simulink model "CellChannels"  (R2024a)
settings: Solver=FixedStepDiscrete  StartTime=0.0  StopTime=10  FixedStep=0.01  RelTol=1e-3
PreLoadFcn:
  | if exist('CellChannels_types', 'file') == 2, CellChannels_types(); end
model workspace (MAT data in the model file):
  CtrlKi_per_s = Simulink.Parameter
  CtrlKi_per_s.Value = 1
  CtrlKi_per_s.Complexity = 'real'
  CtrlKi_per_s.Dimensions = [1 1]
  CtrlKi_per_s.DataType = 'single'
  CtrlKp = Simulink.Parameter
  CtrlKp.Value = 0.2
  CtrlKp.Complexity = 'real'
  CtrlKp.Dimensions = [1 1]
  CtrlKp.DataType = 'single'
  CtrlLimit_V = Simulink.Parameter
  CtrlLimit_V.Value = 0.1
  CtrlLimit_V.Complexity = 'real'
  CtrlLimit_V.Dimensions = [1 1]
  CtrlLimit_V.DataType = 'single'
  OutputFloor_V = Simulink.Parameter
  OutputFloor_V.Value = 0.7
  OutputFloor_V.Complexity = 'real'
  OutputFloor_V.Dimensions = [1 1]
  OutputFloor_V.DataType = 'single'
  OverVoltThd_V = Simulink.Parameter
  OverVoltThd_V.Value = 0.2
  OverVoltThd_V.Complexity = 'real'
  OverVoltThd_V.Dimensions = [1 1]
  OverVoltThd_V.DataType = 'single'
  OverVoltTime_cycles = Simulink.Parameter
  OverVoltTime_cycles.Value = 10
  OverVoltTime_cycles.Complexity = 'real'
  OverVoltTime_cycles.Dimensions = [1 1]
  OverVoltTime_cycles.DataType = 'uint8'
  SetpointLimit_V = Simulink.Parameter
  SetpointLimit_V.Value = 5
  SetpointLimit_V.Complexity = 'real'
  SetpointLimit_V.Dimensions = [1 1]
  SetpointLimit_V.DataType = 'single'
  StepHold_cycles = Simulink.Parameter
  StepHold_cycles.Value = 50
  StepHold_cycles.Complexity = 'real'
  StepHold_cycles.Dimensions = [1 1]
  StepHold_cycles.DataType = 'uint8'
  StepThreshold_V = Simulink.Parameter
  StepThreshold_V.Value = 0.2
  StepThreshold_V.Complexity = 'real'
  StepThreshold_V.Dimensions = [1 1]
  StepThreshold_V.DataType = 'single'
  VoltageSenseFilter = Simulink.Parameter
  VoltageSenseFilter.Value = 0.1
  VoltageSenseFilter.Complexity = 'real'
  VoltageSenseFilter.Dimensions = [1 1]
  VoltageSenseFilter.DataType = 'single'
  VoltageSenseMeas_Ax = Simulink.Parameter
  VoltageSenseMeas_Ax.Value = [0 398.1 795.7 1195.8 1596.4 1996]
  VoltageSenseMeas_Ax.Complexity = 'real'
  VoltageSenseMeas_Ax.Dimensions = [1 6]
  VoltageSenseMeas_Ax.DataType = 'single'
  VoltageSenseValue_T = Simulink.Parameter
  VoltageSenseValue_T.Value = [0 1 2 3 4 5]
  VoltageSenseValue_T.Complexity = 'real'
  VoltageSenseValue_T.Dimensions = [1 6]
  VoltageSenseValue_T.DataType = 'single'
  VoltageSetPwm_T = Simulink.Parameter
  VoltageSetPwm_T.Value = [0 0.185875 0.378085 0.570892 0.763797 0.9566]
  VoltageSetPwm_T.Complexity = 'real'
  VoltageSetPwm_T.Dimensions = [1 6]
  VoltageSetPwm_T.DataType = 'single'
  VoltageSetValue_Ax = Simulink.Parameter
  VoltageSetValue_Ax.Value = [0 1 2 3 4 5]
  VoltageSetValue_Ax.Complexity = 'real'
  VoltageSetValue_Ax.Dimensions = [1 6]
  VoltageSetValue_Ax.DataType = 'single'
values from neighbouring files (symbols this model uses):
  CtrlKi_per_s = 1.0    (= 1)    [CellChannels_data.m]
  CtrlKp = 0.2    [CellChannels_data.m]
  CtrlLimit_V = 0.1    [CellChannels_data.m]
  OutputFloor_V = 0.7    [CellChannels_data.m]
  OverVoltThd_V = 0.2    [CellChannels_data.m]
  OverVoltTime_cycles = 10    [CellChannels_data.m]
  SetpointLimit_V = 5.0    (= 5)    [CellChannels_data.m]
  StepHold_cycles = 50    [CellChannels_data.m]
  StepThreshold_V = 0.2    [CellChannels_data.m]
  VoltageSenseFilter = 0.1    [CellChannels_data.m]
  VoltageSenseMeas_Ax = [0.0 398.1 795.7 1195.8 1596.4 1996.0]    [CellChannels_data.m]
  VoltageSenseValue_T = [0 1 2 3 4 5]    [CellChannels_data.m]
  VoltageSetPwm_T = [0 0.185875 0.378085 0.570892 0.763797 0.9566]    [CellChannels_data.m]
  VoltageSetValue_Ax = [0 1 2 3 4 5]    [CellChannels_data.m]
undefined symbols (not defined in the file or in its folder): QLF_OK
Description:
  | 14 Zellkanaele: Sollwert auf Tastgrad, Freigabe, Istwert, Kalibrierung, Regler und Status
settings Model: ParameterArgumentNames=VoltageSetValue_Ax,VoltageSetPwm_T,VoltageSenseMeas_Ax,VoltageSenseValue_T,SetpointLimit_V,OverVoltThd_V,OverVoltTime_cycles,OutputFloor_V,StepThreshold_V,StepHold_cycles,VoltageSenseFilter,CtrlKp,CtrlKi_per_s,CtrlLimit_V  Creator=danie  LastModifiedBy=danie
settings OptimizationCC: DefaultParameterBehavior=Inlined  EnhancedBackFolding=on  PassReuseOutputArgsAs=Individual arguments  ZeroExternalMemoryAtStartup=off  ZeroInternalMemoryAtStartup=off  OptimizeBlockOrder=speed  DifferentSizesBufferReuse=on  OptimizationCustomize=off  EfficientTunableParamExpr=on
settings DebuggingCC: ParameterTunabilityLossMsg=error
settings HardwareCC: ProdBitPerPointer=32  ProdBitPerSizeT=32  ProdBitPerPtrDiffT=32  ProdLargestAtomicInteger=Long  ProdLargestAtomicFloat=Double  ProdWordSize=32  ProdLongLongMode=on  ProdHWDeviceType=ARM Compatible->ARM Cortex-M
settings SFSimCC: MATLABDynamicMemAlloc=off
settings RTWCC: Description=AUTOSAR  SystemTargetFile=autosar.tlc  GenCodeOnly=on  GenerateMakefile=off  TemplateMakefile=ert_default_tmf  DataTypeReplacement=CDataTypesFixedWidth
settings CodeAppCC: ForceParamTrailComments=on  IgnoreCustomStorageClasses=off  MaxIdLength=63  OperatorAnnotations=on  SimulinkDataObjDesc=on  SFDataObjDesc=on  InsertBlockDesc=on
settings STFCustomTargetCC: MultiwordLength=256  ParMdlRefBuildCompliant=on  CompOptLevelCompliant=on  IncludeMdlTerminateFcn=off  CombineOutputUpdateFcns=on  SuppressErrorStatus=on  ERTCustomFileBanners=on  SupportNonFinite=off  SupportComplex=off  SupportContinuousTime=off  SupportNonInlinedSFcns=off  RemoveResetFunc=on  MATLABClassNameForMDSCustomization=Simulink.SoftwareTarget.ERTCustomization  AutosarCompliant=on  GRTInterface=off  LookupTableObjectStructAxisOrder=2,1,3,4,...  LUTObjectStructOrderEvenSpacing=Size,Table,Breakpoints  SystemTargetFile=autosar.tlc
settings ERTTargetCC: TargetLangStandard=C99 (ISO)  ConcurrentExecutionCompliant=off  IncludeMdlTerminateFcn=off  SuppressErrorStatus=on  SupportNonFinite=off  SupportComplex=off  ModelStepFunctionPrototypeControlCompliant=off  CPPClassGenCompliant=off  AutosarCompliant=on  LookupTableObjectStructAxisOrder=2,1,3,4,...  LUTObjectStructOrderEvenSpacing=Size,Table,Breakpoints  InlinedParameterPlacement=NonHierarchical  ERTCustomFileTemplate=example_file_process.tlc  BooleanTrueId=TRUE  BooleanFalseId=FALSE

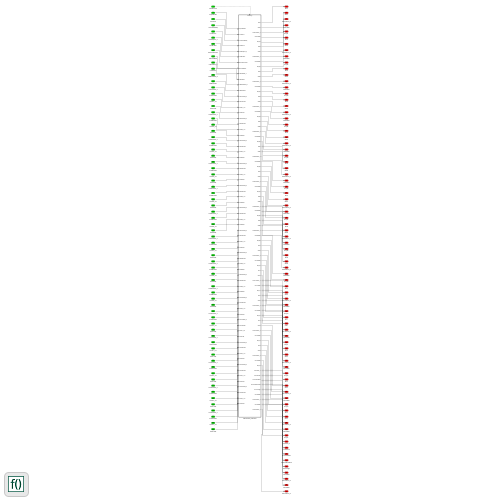
[thumbnail: Simulink's stored preview of the top-level diagram]
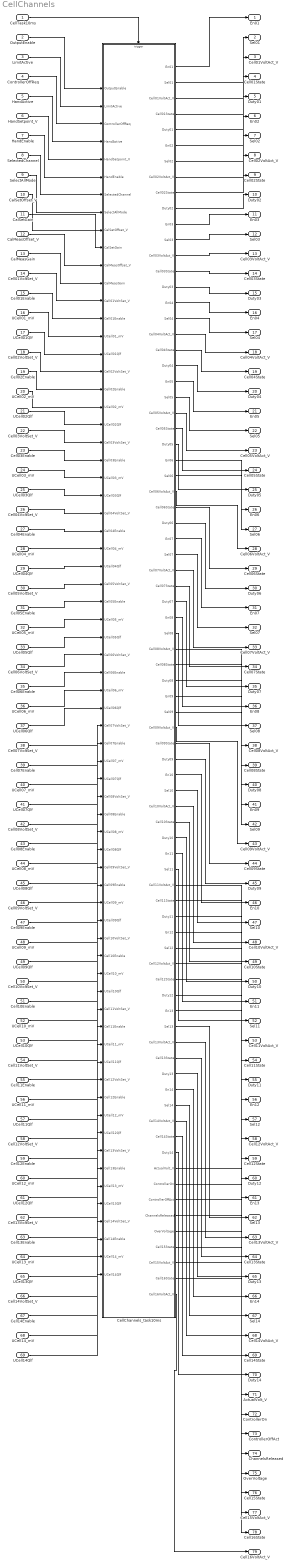
== system CellChannels ==
  CellTask10ms : Inport  SampleTime=0.01  OutputFunctionCall=on
  OutputEnable : Inport  Port=2  OutDataTypeStr=boolean  PortDimensions=1
  LimitActive : Inport  Port=3  OutDataTypeStr=boolean  PortDimensions=1
  ControllerOffReq : Inport  Port=4  OutDataTypeStr=uint8  PortDimensions=1
  HandActive : Inport  Port=5  OutDataTypeStr=boolean  PortDimensions=1
  HandSetpoint_V : Inport  Port=6  OutDataTypeStr=single  PortDimensions=CellCount
  HandEnable : Inport  Port=7  OutDataTypeStr=boolean  PortDimensions=CellCount
  SelectedChannel : Inport  Port=8  OutDataTypeStr=uint8  PortDimensions=1
  SelectAllMode : Inport  Port=9  OutDataTypeStr=boolean  PortDimensions=1
  CalSetOffset_V : Inport  Port=10  OutDataTypeStr=single  PortDimensions=CellCount
  CalSetGain : Inport  Port=11  OutDataTypeStr=single  PortDimensions=CellCount
  CalMeasOffset_V : Inport  Port=12  OutDataTypeStr=single  PortDimensions=CellCount
  CalMeasGain : Inport  Port=13  OutDataTypeStr=single  PortDimensions=CellCount
  Cell01VoltSet_V : Inport  Port=14  OutDataTypeStr=single  PortDimensions=1
  Cell01Enable : Inport  Port=15  OutDataTypeStr=uint8  PortDimensions=1
  UCell01_mV : Inport  Port=16  OutDataTypeStr=uint32  PortDimensions=1
  UCell01Qlf : Inport  Port=17  OutDataTypeStr=uint8  PortDimensions=1
  Cell02VoltSet_V : Inport  Port=18  OutDataTypeStr=single  PortDimensions=1
  Cell02Enable : Inport  Port=19  OutDataTypeStr=uint8  PortDimensions=1
  UCell02_mV : Inport  Port=20  OutDataTypeStr=uint32  PortDimensions=1
  UCell02Qlf : Inport  Port=21  OutDataTypeStr=uint8  PortDimensions=1
  Cell03VoltSet_V : Inport  Port=22  OutDataTypeStr=single  PortDimensions=1
  Cell03Enable : Inport  Port=23  OutDataTypeStr=uint8  PortDimensions=1
  UCell03_mV : Inport  Port=24  OutDataTypeStr=uint32  PortDimensions=1
  UCell03Qlf : Inport  Port=25  OutDataTypeStr=uint8  PortDimensions=1
  Cell04VoltSet_V : Inport  Port=26  OutDataTypeStr=single  PortDimensions=1
  Cell04Enable : Inport  Port=27  OutDataTypeStr=uint8  PortDimensions=1
  UCell04_mV : Inport  Port=28  OutDataTypeStr=uint32  PortDimensions=1
  UCell04Qlf : Inport  Port=29  OutDataTypeStr=uint8  PortDimensions=1
  Cell05VoltSet_V : Inport  Port=30  OutDataTypeStr=single  PortDimensions=1
  Cell05Enable : Inport  Port=31  OutDataTypeStr=uint8  PortDimensions=1
  UCell05_mV : Inport  Port=32  OutDataTypeStr=uint32  PortDimensions=1
  UCell05Qlf : Inport  Port=33  OutDataTypeStr=uint8  PortDimensions=1
  Cell06VoltSet_V : Inport  Port=34  OutDataTypeStr=single  PortDimensions=1
  Cell06Enable : Inport  Port=35  OutDataTypeStr=uint8  PortDimensions=1
  UCell06_mV : Inport  Port=36  OutDataTypeStr=uint32  PortDimensions=1
  UCell06Qlf : Inport  Port=37  OutDataTypeStr=uint8  PortDimensions=1
  Cell07VoltSet_V : Inport  Port=38  OutDataTypeStr=single  PortDimensions=1
  Cell07Enable : Inport  Port=39  OutDataTypeStr=uint8  PortDimensions=1
  UCell07_mV : Inport  Port=40  OutDataTypeStr=uint32  PortDimensions=1
  UCell07Qlf : Inport  Port=41  OutDataTypeStr=uint8  PortDimensions=1
  Cell08VoltSet_V : Inport  Port=42  OutDataTypeStr=single  PortDimensions=1
  Cell08Enable : Inport  Port=43  OutDataTypeStr=uint8  PortDimensions=1
  UCell08_mV : Inport  Port=44  OutDataTypeStr=uint32  PortDimensions=1
  UCell08Qlf : Inport  Port=45  OutDataTypeStr=uint8  PortDimensions=1
  Cell09VoltSet_V : Inport  Port=46  OutDataTypeStr=single  PortDimensions=1
  Cell09Enable : Inport  Port=47  OutDataTypeStr=uint8  PortDimensions=1
  UCell09_mV : Inport  Port=48  OutDataTypeStr=uint32  PortDimensions=1
  UCell09Qlf : Inport  Port=49  OutDataTypeStr=uint8  PortDimensions=1
  Cell10VoltSet_V : Inport  Port=50  OutDataTypeStr=single  PortDimensions=1
  Cell10Enable : Inport  Port=51  OutDataTypeStr=uint8  PortDimensions=1
  UCell10_mV : Inport  Port=52  OutDataTypeStr=uint32  PortDimensions=1
  UCell10Qlf : Inport  Port=53  OutDataTypeStr=uint8  PortDimensions=1
  Cell11VoltSet_V : Inport  Port=54  OutDataTypeStr=single  PortDimensions=1
  Cell11Enable : Inport  Port=55  OutDataTypeStr=uint8  PortDimensions=1
  UCell11_mV : Inport  Port=56  OutDataTypeStr=uint32  PortDimensions=1
  UCell11Qlf : Inport  Port=57  OutDataTypeStr=uint8  PortDimensions=1
  Cell12VoltSet_V : Inport  Port=58  OutDataTypeStr=single  PortDimensions=1
  Cell12Enable : Inport  Port=59  OutDataTypeStr=uint8  PortDimensions=1
  UCell12_mV : Inport  Port=60  OutDataTypeStr=uint32  PortDimensions=1
  UCell12Qlf : Inport  Port=61  OutDataTypeStr=uint8  PortDimensions=1
  Cell13VoltSet_V : Inport  Port=62  OutDataTypeStr=single  PortDimensions=1
  Cell13Enable : Inport  Port=63  OutDataTypeStr=uint8  PortDimensions=1
  UCell13_mV : Inport  Port=64  OutDataTypeStr=uint32  PortDimensions=1
  UCell13Qlf : Inport  Port=65  OutDataTypeStr=uint8  PortDimensions=1
  Cell14VoltSet_V : Inport  Port=66  OutDataTypeStr=single  PortDimensions=1
  Cell14Enable : Inport  Port=67  OutDataTypeStr=uint8  PortDimensions=1
  UCell14_mV : Inport  Port=68  OutDataTypeStr=uint32  PortDimensions=1
  UCell14Qlf : Inport  Port=69  OutDataTypeStr=uint8  PortDimensions=1
  CellChannels_task10ms : Subsystem  TreatAsAtomicUnit=on
  En01 : Outport  OutDataTypeStr=boolean  PortDimensions=1
  Sel01 : Outport  Port=2  OutDataTypeStr=boolean  PortDimensions=1
  Cell01VoltAct_V : Outport  Port=3  OutDataTypeStr=single  PortDimensions=1
  Cell01State : Outport  Port=4  OutDataTypeStr=uint8  PortDimensions=1
  Duty01 : Outport  Port=5  OutDataTypeStr=uint16  PortDimensions=1
  En02 : Outport  Port=6  OutDataTypeStr=boolean  PortDimensions=1
  Sel02 : Outport  Port=7  OutDataTypeStr=boolean  PortDimensions=1
  Cell02VoltAct_V : Outport  Port=8  OutDataTypeStr=single  PortDimensions=1
  Cell02State : Outport  Port=9  OutDataTypeStr=uint8  PortDimensions=1
  Duty02 : Outport  Port=10  OutDataTypeStr=uint16  PortDimensions=1
  En03 : Outport  Port=11  OutDataTypeStr=boolean  PortDimensions=1
  Sel03 : Outport  Port=12  OutDataTypeStr=boolean  PortDimensions=1
  Cell03VoltAct_V : Outport  Port=13  OutDataTypeStr=single  PortDimensions=1
  Cell03State : Outport  Port=14  OutDataTypeStr=uint8  PortDimensions=1
  Duty03 : Outport  Port=15  OutDataTypeStr=uint16  PortDimensions=1
  En04 : Outport  Port=16  OutDataTypeStr=boolean  PortDimensions=1
  Sel04 : Outport  Port=17  OutDataTypeStr=boolean  PortDimensions=1
  Cell04VoltAct_V : Outport  Port=18  OutDataTypeStr=single  PortDimensions=1
  Cell04State : Outport  Port=19  OutDataTypeStr=uint8  PortDimensions=1
  Duty04 : Outport  Port=20  OutDataTypeStr=uint16  PortDimensions=1
  En05 : Outport  Port=21  OutDataTypeStr=boolean  PortDimensions=1
  Sel05 : Outport  Port=22  OutDataTypeStr=boolean  PortDimensions=1
  Cell05VoltAct_V : Outport  Port=23  OutDataTypeStr=single  PortDimensions=1
  Cell05State : Outport  Port=24  OutDataTypeStr=uint8  PortDimensions=1
  Duty05 : Outport  Port=25  OutDataTypeStr=uint16  PortDimensions=1
  En06 : Outport  Port=26  OutDataTypeStr=boolean  PortDimensions=1
  Sel06 : Outport  Port=27  OutDataTypeStr=boolean  PortDimensions=1
  Cell06VoltAct_V : Outport  Port=28  OutDataTypeStr=single  PortDimensions=1
  Cell06State : Outport  Port=29  OutDataTypeStr=uint8  PortDimensions=1
  Duty06 : Outport  Port=30  OutDataTypeStr=uint16  PortDimensions=1
  En07 : Outport  Port=31  OutDataTypeStr=boolean  PortDimensions=1
  Sel07 : Outport  Port=32  OutDataTypeStr=boolean  PortDimensions=1
  Cell07VoltAct_V : Outport  Port=33  OutDataTypeStr=single  PortDimensions=1
  Cell07State : Outport  Port=34  OutDataTypeStr=uint8  PortDimensions=1
  Duty07 : Outport  Port=35  OutDataTypeStr=uint16  PortDimensions=1
  En08 : Outport  Port=36  OutDataTypeStr=boolean  PortDimensions=1
  Sel08 : Outport  Port=37  OutDataTypeStr=boolean  PortDimensions=1
  Cell08VoltAct_V : Outport  Port=38  OutDataTypeStr=single  PortDimensions=1
  Cell08State : Outport  Port=39  OutDataTypeStr=uint8  PortDimensions=1
  Duty08 : Outport  Port=40  OutDataTypeStr=uint16  PortDimensions=1
  En09 : Outport  Port=41  OutDataTypeStr=boolean  PortDimensions=1
  Sel09 : Outport  Port=42  OutDataTypeStr=boolean  PortDimensions=1
  Cell09VoltAct_V : Outport  Port=43  OutDataTypeStr=single  PortDimensions=1
  Cell09State : Outport  Port=44  OutDataTypeStr=uint8  PortDimensions=1
  Duty09 : Outport  Port=45  OutDataTypeStr=uint16  PortDimensions=1
  En10 : Outport  Port=46  OutDataTypeStr=boolean  PortDimensions=1
  Sel10 : Outport  Port=47  OutDataTypeStr=boolean  PortDimensions=1
  Cell10VoltAct_V : Outport  Port=48  OutDataTypeStr=single  PortDimensions=1
  Cell10State : Outport  Port=49  OutDataTypeStr=uint8  PortDimensions=1
  Duty10 : Outport  Port=50  OutDataTypeStr=uint16  PortDimensions=1
  En11 : Outport  Port=51  OutDataTypeStr=boolean  PortDimensions=1
  Sel11 : Outport  Port=52  OutDataTypeStr=boolean  PortDimensions=1
  Cell11VoltAct_V : Outport  Port=53  OutDataTypeStr=single  PortDimensions=1
  Cell11State : Outport  Port=54  OutDataTypeStr=uint8  PortDimensions=1
  Duty11 : Outport  Port=55  OutDataTypeStr=uint16  PortDimensions=1
  En12 : Outport  Port=56  OutDataTypeStr=boolean  PortDimensions=1
  Sel12 : Outport  Port=57  OutDataTypeStr=boolean  PortDimensions=1
  Cell12VoltAct_V : Outport  Port=58  OutDataTypeStr=single  PortDimensions=1
  Cell12State : Outport  Port=59  OutDataTypeStr=uint8  PortDimensions=1
  Duty12 : Outport  Port=60  OutDataTypeStr=uint16  PortDimensions=1
  En13 : Outport  Port=61  OutDataTypeStr=boolean  PortDimensions=1
  Sel13 : Outport  Port=62  OutDataTypeStr=boolean  PortDimensions=1
  Cell13VoltAct_V : Outport  Port=63  OutDataTypeStr=single  PortDimensions=1
  Cell13State : Outport  Port=64  OutDataTypeStr=uint8  PortDimensions=1
  Duty13 : Outport  Port=65  OutDataTypeStr=uint16  PortDimensions=1
  En14 : Outport  Port=66  OutDataTypeStr=boolean  PortDimensions=1
  Sel14 : Outport  Port=67  OutDataTypeStr=boolean  PortDimensions=1
  Cell14VoltAct_V : Outport  Port=68  OutDataTypeStr=single  PortDimensions=1
  Cell14State : Outport  Port=69  OutDataTypeStr=uint8  PortDimensions=1
  Duty14 : Outport  Port=70  OutDataTypeStr=uint16  PortDimensions=1
  ActualVolt_V : Outport  Port=71  OutDataTypeStr=single  PortDimensions=CellCount
  ControllerOn : Outport  Port=72  OutDataTypeStr=boolean  PortDimensions=1
  ControllerOffAct : Outport  Port=73  OutDataTypeStr=uint8  PortDimensions=1
  ChannelsReleased : Outport  Port=74  OutDataTypeStr=boolean  PortDimensions=1
  OverVoltage : Outport  Port=75  OutDataTypeStr=boolean  PortDimensions=1
  Cell15State : Outport  Port=76  OutDataTypeStr=uint8  PortDimensions=1
  Cell15VoltAct_V : Outport  Port=77  OutDataTypeStr=single  PortDimensions=1
  Cell16State : Outport  Port=78  OutDataTypeStr=uint8  PortDimensions=1
  Cell16VoltAct_V : Outport  Port=79  OutDataTypeStr=single  PortDimensions=1
  wires:
  CellTask10ms/1 -> CellChannels_task10ms/Trigger
  OutputEnable/1 -> CellChannels_task10ms/1(OutputEnable)
  LimitActive/1 -> CellChannels_task10ms/2(LimitActive)
  ControllerOffReq/1 -> CellChannels_task10ms/3(ControllerOffReq)
  HandActive/1 -> CellChannels_task10ms/4(HandActive)
  HandSetpoint_V/1 -> CellChannels_task10ms/5(HandSetpoint_V)
  HandEnable/1 -> CellChannels_task10ms/6(HandEnable)
  SelectedChannel/1 -> CellChannels_task10ms/7(SelectedChannel)
  SelectAllMode/1 -> CellChannels_task10ms/8(SelectAllMode)
  CalSetOffset_V/1 -> CellChannels_task10ms/9(CalSetOffset_V)
  CalSetGain/1 -> CellChannels_task10ms/10(CalSetGain)
  CalMeasOffset_V/1 -> CellChannels_task10ms/11(CalMeasOffset_V)
  CalMeasGain/1 -> CellChannels_task10ms/12(CalMeasGain)
  Cell01VoltSet_V/1 -> CellChannels_task10ms/13(Cell01VoltSet_V)
  Cell01Enable/1 -> CellChannels_task10ms/14(Cell01Enable)
  UCell01_mV/1 -> CellChannels_task10ms/15(UCell01_mV)
  UCell01Qlf/1 -> CellChannels_task10ms/16(UCell01Qlf)
  Cell02VoltSet_V/1 -> CellChannels_task10ms/17(Cell02VoltSet_V)
  Cell02Enable/1 -> CellChannels_task10ms/18(Cell02Enable)
  UCell02_mV/1 -> CellChannels_task10ms/19(UCell02_mV)
  UCell02Qlf/1 -> CellChannels_task10ms/20(UCell02Qlf)
  Cell03VoltSet_V/1 -> CellChannels_task10ms/21(Cell03VoltSet_V)
  Cell03Enable/1 -> CellChannels_task10ms/22(Cell03Enable)
  UCell03_mV/1 -> CellChannels_task10ms/23(UCell03_mV)
  UCell03Qlf/1 -> CellChannels_task10ms/24(UCell03Qlf)
  Cell04VoltSet_V/1 -> CellChannels_task10ms/25(Cell04VoltSet_V)
  Cell04Enable/1 -> CellChannels_task10ms/26(Cell04Enable)
  UCell04_mV/1 -> CellChannels_task10ms/27(UCell04_mV)
  UCell04Qlf/1 -> CellChannels_task10ms/28(UCell04Qlf)
  Cell05VoltSet_V/1 -> CellChannels_task10ms/29(Cell05VoltSet_V)
  Cell05Enable/1 -> CellChannels_task10ms/30(Cell05Enable)
  UCell05_mV/1 -> CellChannels_task10ms/31(UCell05_mV)
  UCell05Qlf/1 -> CellChannels_task10ms/32(UCell05Qlf)
  Cell06VoltSet_V/1 -> CellChannels_task10ms/33(Cell06VoltSet_V)
  Cell06Enable/1 -> CellChannels_task10ms/34(Cell06Enable)
  UCell06_mV/1 -> CellChannels_task10ms/35(UCell06_mV)
  UCell06Qlf/1 -> CellChannels_task10ms/36(UCell06Qlf)
  Cell07VoltSet_V/1 -> CellChannels_task10ms/37(Cell07VoltSet_V)
  Cell07Enable/1 -> CellChannels_task10ms/38(Cell07Enable)
  UCell07_mV/1 -> CellChannels_task10ms/39(UCell07_mV)
  UCell07Qlf/1 -> CellChannels_task10ms/40(UCell07Qlf)
  Cell08VoltSet_V/1 -> CellChannels_task10ms/41(Cell08VoltSet_V)
  Cell08Enable/1 -> CellChannels_task10ms/42(Cell08Enable)
  UCell08_mV/1 -> CellChannels_task10ms/43(UCell08_mV)
  UCell08Qlf/1 -> CellChannels_task10ms/44(UCell08Qlf)
  Cell09VoltSet_V/1 -> CellChannels_task10ms/45(Cell09VoltSet_V)
  Cell09Enable/1 -> CellChannels_task10ms/46(Cell09Enable)
  UCell09_mV/1 -> CellChannels_task10ms/47(UCell09_mV)
  UCell09Qlf/1 -> CellChannels_task10ms/48(UCell09Qlf)
  Cell10VoltSet_V/1 -> CellChannels_task10ms/49(Cell10VoltSet_V)
  Cell10Enable/1 -> CellChannels_task10ms/50(Cell10Enable)
  UCell10_mV/1 -> CellChannels_task10ms/51(UCell10_mV)
  UCell10Qlf/1 -> CellChannels_task10ms/52(UCell10Qlf)
  Cell11VoltSet_V/1 -> CellChannels_task10ms/53(Cell11VoltSet_V)
  Cell11Enable/1 -> CellChannels_task10ms/54(Cell11Enable)
  UCell11_mV/1 -> CellChannels_task10ms/55(UCell11_mV)
  UCell11Qlf/1 -> CellChannels_task10ms/56(UCell11Qlf)
  Cell12VoltSet_V/1 -> CellChannels_task10ms/57(Cell12VoltSet_V)
  Cell12Enable/1 -> CellChannels_task10ms/58(Cell12Enable)
  UCell12_mV/1 -> CellChannels_task10ms/59(UCell12_mV)
  UCell12Qlf/1 -> CellChannels_task10ms/60(UCell12Qlf)
  Cell13VoltSet_V/1 -> CellChannels_task10ms/61(Cell13VoltSet_V)
  Cell13Enable/1 -> CellChannels_task10ms/62(Cell13Enable)
  UCell13_mV/1 -> CellChannels_task10ms/63(UCell13_mV)
  UCell13Qlf/1 -> CellChannels_task10ms/64(UCell13Qlf)
  Cell14VoltSet_V/1 -> CellChannels_task10ms/65(Cell14VoltSet_V)
  Cell14Enable/1 -> CellChannels_task10ms/66(Cell14Enable)
  UCell14_mV/1 -> CellChannels_task10ms/67(UCell14_mV)
  UCell14Qlf/1 -> CellChannels_task10ms/68(UCell14Qlf)
  CellChannels_task10ms/1(En01) -> En01/1
  CellChannels_task10ms/2(Sel01) -> Sel01/1
  CellChannels_task10ms/3(Cell01VoltAct_V) -> Cell01VoltAct_V/1
  CellChannels_task10ms/4(Cell01State) -> Cell01State/1
  CellChannels_task10ms/5(Duty01) -> Duty01/1
  CellChannels_task10ms/6(En02) -> En02/1
  CellChannels_task10ms/7(Sel02) -> Sel02/1
  CellChannels_task10ms/8(Cell02VoltAct_V) -> Cell02VoltAct_V/1
  CellChannels_task10ms/9(Cell02State) -> Cell02State/1
  CellChannels_task10ms/10(Duty02) -> Duty02/1
  CellChannels_task10ms/11(En03) -> En03/1
  CellChannels_task10ms/12(Sel03) -> Sel03/1
  CellChannels_task10ms/13(Cell03VoltAct_V) -> Cell03VoltAct_V/1
  CellChannels_task10ms/14(Cell03State) -> Cell03State/1
  CellChannels_task10ms/15(Duty03) -> Duty03/1
  CellChannels_task10ms/16(En04) -> En04/1
  CellChannels_task10ms/17(Sel04) -> Sel04/1
  CellChannels_task10ms/18(Cell04VoltAct_V) -> Cell04VoltAct_V/1
  CellChannels_task10ms/19(Cell04State) -> Cell04State/1
  CellChannels_task10ms/20(Duty04) -> Duty04/1
  CellChannels_task10ms/21(En05) -> En05/1
  CellChannels_task10ms/22(Sel05) -> Sel05/1
  CellChannels_task10ms/23(Cell05VoltAct_V) -> Cell05VoltAct_V/1
  CellChannels_task10ms/24(Cell05State) -> Cell05State/1
  CellChannels_task10ms/25(Duty05) -> Duty05/1
  CellChannels_task10ms/26(En06) -> En06/1
  CellChannels_task10ms/27(Sel06) -> Sel06/1
  CellChannels_task10ms/28(Cell06VoltAct_V) -> Cell06VoltAct_V/1
  CellChannels_task10ms/29(Cell06State) -> Cell06State/1
  CellChannels_task10ms/30(Duty06) -> Duty06/1
  CellChannels_task10ms/31(En07) -> En07/1
  CellChannels_task10ms/32(Sel07) -> Sel07/1
  CellChannels_task10ms/33(Cell07VoltAct_V) -> Cell07VoltAct_V/1
  CellChannels_task10ms/34(Cell07State) -> Cell07State/1
  CellChannels_task10ms/35(Duty07) -> Duty07/1
  CellChannels_task10ms/36(En08) -> En08/1
  CellChannels_task10ms/37(Sel08) -> Sel08/1
  CellChannels_task10ms/38(Cell08VoltAct_V) -> Cell08VoltAct_V/1
  CellChannels_task10ms/39(Cell08State) -> Cell08State/1
  CellChannels_task10ms/40(Duty08) -> Duty08/1
  CellChannels_task10ms/41(En09) -> En09/1
  CellChannels_task10ms/42(Sel09) -> Sel09/1
  CellChannels_task10ms/43(Cell09VoltAct_V) -> Cell09VoltAct_V/1
  CellChannels_task10ms/44(Cell09State) -> Cell09State/1
  CellChannels_task10ms/45(Duty09) -> Duty09/1
  CellChannels_task10ms/46(En10) -> En10/1
  CellChannels_task10ms/47(Sel10) -> Sel10/1
  CellChannels_task10ms/48(Cell10VoltAct_V) -> Cell10VoltAct_V/1
  CellChannels_task10ms/49(Cell10State) -> Cell10State/1
  CellChannels_task10ms/50(Duty10) -> Duty10/1
  CellChannels_task10ms/51(En11) -> En11/1
  CellChannels_task10ms/52(Sel11) -> Sel11/1
  CellChannels_task10ms/53(Cell11VoltAct_V) -> Cell11VoltAct_V/1
  CellChannels_task10ms/54(Cell11State) -> Cell11State/1
  CellChannels_task10ms/55(Duty11) -> Duty11/1
  CellChannels_task10ms/56(En12) -> En12/1
  CellChannels_task10ms/57(Sel12) -> Sel12/1
  CellChannels_task10ms/58(Cell12VoltAct_V) -> Cell12VoltAct_V/1
  CellChannels_task10ms/59(Cell12State) -> Cell12State/1
  CellChannels_task10ms/60(Duty12) -> Duty12/1
  CellChannels_task10ms/61(En13) -> En13/1
  CellChannels_task10ms/62(Sel13) -> Sel13/1
  CellChannels_task10ms/63(Cell13VoltAct_V) -> Cell13VoltAct_V/1
  CellChannels_task10ms/64(Cell13State) -> Cell13State/1
  CellChannels_task10ms/65(Duty13) -> Duty13/1
  CellChannels_task10ms/66(En14) -> En14/1
  CellChannels_task10ms/67(Sel14) -> Sel14/1
  CellChannels_task10ms/68(Cell14VoltAct_V) -> Cell14VoltAct_V/1
  CellChannels_task10ms/69(Cell14State) -> Cell14State/1
  CellChannels_task10ms/70(Duty14) -> Duty14/1
  CellChannels_task10ms/71(ActualVolt_V) -> ActualVolt_V/1
  CellChannels_task10ms/72(ControllerOn) -> ControllerOn/1
  CellChannels_task10ms/73(ControllerOffAct) -> ControllerOffAct/1
  CellChannels_task10ms/74(ChannelsReleased) -> ChannelsReleased/1
  CellChannels_task10ms/75(OverVoltage) -> OverVoltage/1
  CellChannels_task10ms/76(Cell15State) -> Cell15State/1
  CellChannels_task10ms/77(Cell15VoltAct_V) -> Cell15VoltAct_V/1
  CellChannels_task10ms/78(Cell16State) -> Cell16State/1
  CellChannels_task10ms/79(Cell16VoltAct_V) -> Cell16VoltAct_V/1

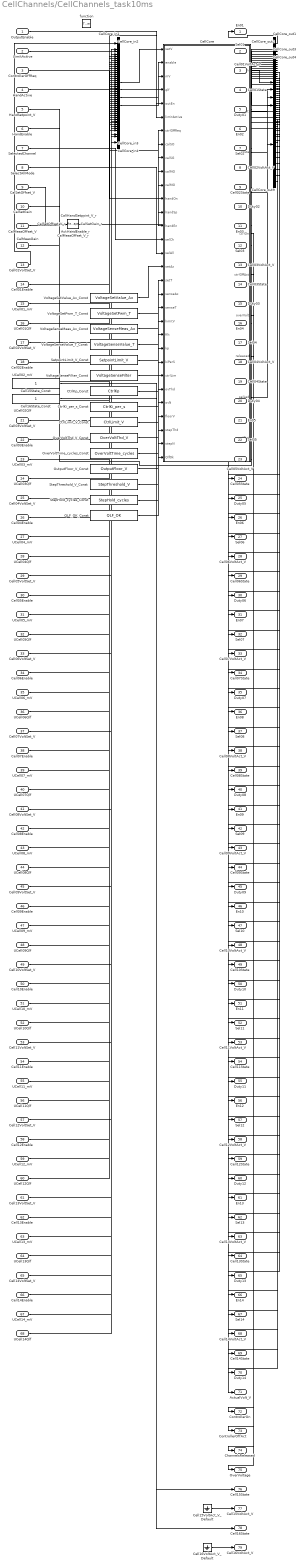
== system CellChannels/CellChannels_task10ms ==
  OutputEnable : Inport
  LimitActive : Inport  Port=2
  ControllerOffReq : Inport  Port=3
  HandActive : Inport  Port=4
  HandSetpoint_V : Inport  Port=5
  HandEnable : Inport  Port=6
  SelectedChannel : Inport  Port=7
  SelectAllMode : Inport  Port=8
  CalSetOffset_V : Inport  Port=9
  CalSetGain : Inport  Port=10
  CalMeasOffset_V : Inport  Port=11
  CalMeasGain : Inport  Port=12
  Cell01VoltSet_V : Inport  Port=13
  Cell01Enable : Inport  Port=14
  UCell01_mV : Inport  Port=15
  UCell01Qlf : Inport  Port=16
  Cell02VoltSet_V : Inport  Port=17
  Cell02Enable : Inport  Port=18
  UCell02_mV : Inport  Port=19
  UCell02Qlf : Inport  Port=20
  Cell03VoltSet_V : Inport  Port=21
  Cell03Enable : Inport  Port=22
  UCell03_mV : Inport  Port=23
  UCell03Qlf : Inport  Port=24
  Cell04VoltSet_V : Inport  Port=25
  Cell04Enable : Inport  Port=26
  UCell04_mV : Inport  Port=27
  UCell04Qlf : Inport  Port=28
  Cell05VoltSet_V : Inport  Port=29
  Cell05Enable : Inport  Port=30
  UCell05_mV : Inport  Port=31
  UCell05Qlf : Inport  Port=32
  Cell06VoltSet_V : Inport  Port=33
  Cell06Enable : Inport  Port=34
  UCell06_mV : Inport  Port=35
  UCell06Qlf : Inport  Port=36
  Cell07VoltSet_V : Inport  Port=37
  Cell07Enable : Inport  Port=38
  UCell07_mV : Inport  Port=39
  UCell07Qlf : Inport  Port=40
  Cell08VoltSet_V : Inport  Port=41
  Cell08Enable : Inport  Port=42
  UCell08_mV : Inport  Port=43
  UCell08Qlf : Inport  Port=44
  Cell09VoltSet_V : Inport  Port=45
  Cell09Enable : Inport  Port=46
  UCell09_mV : Inport  Port=47
  UCell09Qlf : Inport  Port=48
  Cell10VoltSet_V : Inport  Port=49
  Cell10Enable : Inport  Port=50
  UCell10_mV : Inport  Port=51
  UCell10Qlf : Inport  Port=52
  Cell11VoltSet_V : Inport  Port=53
  Cell11Enable : Inport  Port=54
  UCell11_mV : Inport  Port=55
  UCell11Qlf : Inport  Port=56
  Cell12VoltSet_V : Inport  Port=57
  Cell12Enable : Inport  Port=58
  UCell12_mV : Inport  Port=59
  UCell12Qlf : Inport  Port=60
  Cell13VoltSet_V : Inport  Port=61
  Cell13Enable : Inport  Port=62
  UCell13_mV : Inport  Port=63
  UCell13Qlf : Inport  Port=64
  Cell14VoltSet_V : Inport  Port=65
  Cell14Enable : Inport  Port=66
  UCell14_mV : Inport  Port=67
  UCell14Qlf : Inport  Port=68
  function : TriggerPort  TriggerType=function-call  VariantControl=(inherit)  SampleTimeType=periodic  SampleTime=0.01
  ActualVolt_V_r : Reshape
  CalMeasGain_r : Reshape  OutputDimensionality=Customize  OutputDimensions=[14 1]
  CalMeasOffset_V_r : Reshape  OutputDimensionality=Customize  OutputDimensions=[14 1]
  CalSetGain_r : Reshape  OutputDimensionality=Customize  OutputDimensions=[14 1]
  CalSetOffset_V_r : Reshape  OutputDimensionality=Customize  OutputDimensions=[14 1]
  Cell15State_Const : Constant  OutDataTypeStr=uint8
  Cell15VoltAct_V_Default : Ground
  Cell16State_Const : Constant  OutDataTypeStr=uint8
  Cell16VoltAct_V_Default : Ground
  CellCore : MATLAB Function  TreatAsAtomicUnit=on
  CellCore_in{1..4} (4 alike) : Mux  Inputs=14
  CellCore_out{1..4,9} (5 alike) : Demux  Outputs=14
  CtrlKi_per_s_Const : Constant  Value=CtrlKi_per_s  OutDataTypeStr=single
  CtrlKp_Const : Constant  Value=CtrlKp  OutDataTypeStr=single
  CtrlLimit_V_Const : Constant  Value=CtrlLimit_V  OutDataTypeStr=single
  HandEnable_r : Reshape  OutputDimensionality=Customize  OutputDimensions=[14 1]
  HandSetpoint_V_r : Reshape  OutputDimensionality=Customize  OutputDimensions=[14 1]
  OutputFloor_V_Const : Constant  Value=OutputFloor_V  OutDataTypeStr=single
  OverVoltThd_V_Const : Constant  Value=OverVoltThd_V  OutDataTypeStr=single
  OverVoltTime_cycles_Const : Constant  Value=OverVoltTime_cycles  OutDataTypeStr=uint8
  QLF_OK_Const : Constant  Value=QLF_OK  OutDataTypeStr=uint8
  SetpointLimit_V_Const : Constant  Value=SetpointLimit_V  OutDataTypeStr=single
  StepHold_cycles_Const : Constant  Value=StepHold_cycles  OutDataTypeStr=uint8
  StepThreshold_V_Const : Constant  Value=StepThreshold_V  OutDataTypeStr=single
  VoltageSenseFilter_Const : Constant  Value=VoltageSenseFilter  OutDataTypeStr=single
  VoltageSenseMeas_Ax_Const : Constant  Value=VoltageSenseMeas_Ax  OutDataTypeStr=single
  VoltageSenseValue_T_Const : Constant  Value=VoltageSenseValue_T  OutDataTypeStr=single
  VoltageSetPwm_T_Const : Constant  Value=VoltageSetPwm_T  OutDataTypeStr=single
  VoltageSetValue_Ax_Const : Constant  Value=VoltageSetValue_Ax  OutDataTypeStr=single
  En01 : Outport
  Sel01 : Outport  Port=2
  Cell01VoltAct_V : Outport  Port=3
  Cell01State : Outport  Port=4
  Duty01 : Outport  Port=5
  En02 : Outport  Port=6
  Sel02 : Outport  Port=7
  Cell02VoltAct_V : Outport  Port=8
  Cell02State : Outport  Port=9
  Duty02 : Outport  Port=10
  En03 : Outport  Port=11
  Sel03 : Outport  Port=12
  Cell03VoltAct_V : Outport  Port=13
  Cell03State : Outport  Port=14
  Duty03 : Outport  Port=15
  En04 : Outport  Port=16
  Sel04 : Outport  Port=17
  Cell04VoltAct_V : Outport  Port=18
  Cell04State : Outport  Port=19
  Duty04 : Outport  Port=20
  En05 : Outport  Port=21
  Sel05 : Outport  Port=22
  Cell05VoltAct_V : Outport  Port=23
  Cell05State : Outport  Port=24
  Duty05 : Outport  Port=25
  En06 : Outport  Port=26
  Sel06 : Outport  Port=27
  Cell06VoltAct_V : Outport  Port=28
  Cell06State : Outport  Port=29
  Duty06 : Outport  Port=30
  En07 : Outport  Port=31
  Sel07 : Outport  Port=32
  Cell07VoltAct_V : Outport  Port=33
  Cell07State : Outport  Port=34
  Duty07 : Outport  Port=35
  En08 : Outport  Port=36
  Sel08 : Outport  Port=37
  Cell08VoltAct_V : Outport  Port=38
  Cell08State : Outport  Port=39
  Duty08 : Outport  Port=40
  En09 : Outport  Port=41
  Sel09 : Outport  Port=42
  Cell09VoltAct_V : Outport  Port=43
  Cell09State : Outport  Port=44
  Duty09 : Outport  Port=45
  En10 : Outport  Port=46
  Sel10 : Outport  Port=47
  Cell10VoltAct_V : Outport  Port=48
  Cell10State : Outport  Port=49
  Duty10 : Outport  Port=50
  En11 : Outport  Port=51
  Sel11 : Outport  Port=52
  Cell11VoltAct_V : Outport  Port=53
  Cell11State : Outport  Port=54
  Duty11 : Outport  Port=55
  En12 : Outport  Port=56
  Sel12 : Outport  Port=57
  Cell12VoltAct_V : Outport  Port=58
  Cell12State : Outport  Port=59
  Duty12 : Outport  Port=60
  En13 : Outport  Port=61
  Sel13 : Outport  Port=62
  Cell13VoltAct_V : Outport  Port=63
  Cell13State : Outport  Port=64
  Duty13 : Outport  Port=65
  En14 : Outport  Port=66
  Sel14 : Outport  Port=67
  Cell14VoltAct_V : Outport  Port=68
  Cell14State : Outport  Port=69
  Duty14 : Outport  Port=70
  ActualVolt_V : Outport  Port=71
  ControllerOn : Outport  Port=72
  ControllerOffAct : Outport  Port=73
  ChannelsReleased : Outport  Port=74
  OverVoltage : Outport  Port=75
  Cell15State : Outport  Port=76
  Cell15VoltAct_V : Outport  Port=77
  Cell16State : Outport  Port=78
  Cell16VoltAct_V : Outport  Port=79
  wires:
  CalSetOffset_V/1 -> CalSetOffset_V_r/1
  CalSetGain/1 -> CalSetGain_r/1
  CalMeasOffset_V/1 -> CalMeasOffset_V_r/1
  CalMeasGain/1 -> CalMeasGain_r/1
  HandSetpoint_V/1 -> HandSetpoint_V_r/1
  HandEnable/1 -> HandEnable_r/1
  ActualVolt_V_r/1 -> ActualVolt_V/1
  Cell01VoltSet_V/1 -> CellCore_in1/1
  Cell02VoltSet_V/1 -> CellCore_in1/2
  Cell03VoltSet_V/1 -> CellCore_in1/3
  Cell04VoltSet_V/1 -> CellCore_in1/4
  Cell05VoltSet_V/1 -> CellCore_in1/5
  Cell06VoltSet_V/1 -> CellCore_in1/6
  Cell07VoltSet_V/1 -> CellCore_in1/7
  Cell08VoltSet_V/1 -> CellCore_in1/8
  Cell09VoltSet_V/1 -> CellCore_in1/9
  Cell10VoltSet_V/1 -> CellCore_in1/10
  Cell11VoltSet_V/1 -> CellCore_in1/11
  Cell12VoltSet_V/1 -> CellCore_in1/12
  Cell13VoltSet_V/1 -> CellCore_in1/13
  Cell14VoltSet_V/1 -> CellCore_in1/14
  CellCore_in1/1 -> CellCore/1(setV)
  Cell01Enable/1 -> CellCore_in2/1
  Cell02Enable/1 -> CellCore_in2/2
  Cell03Enable/1 -> CellCore_in2/3
  Cell04Enable/1 -> CellCore_in2/4
  Cell05Enable/1 -> CellCore_in2/5
  Cell06Enable/1 -> CellCore_in2/6
  Cell07Enable/1 -> CellCore_in2/7
  Cell08Enable/1 -> CellCore_in2/8
  Cell09Enable/1 -> CellCore_in2/9
  Cell10Enable/1 -> CellCore_in2/10
  Cell11Enable/1 -> CellCore_in2/11
  Cell12Enable/1 -> CellCore_in2/12
  Cell13Enable/1 -> CellCore_in2/13
  Cell14Enable/1 -> CellCore_in2/14
  CellCore_in2/1 -> CellCore/2(enable)
  UCell01_mV/1 -> CellCore_in3/1
  UCell02_mV/1 -> CellCore_in3/2
  UCell03_mV/1 -> CellCore_in3/3
  UCell04_mV/1 -> CellCore_in3/4
  UCell05_mV/1 -> CellCore_in3/5
  UCell06_mV/1 -> CellCore_in3/6
  UCell07_mV/1 -> CellCore_in3/7
  UCell08_mV/1 -> CellCore_in3/8
  UCell09_mV/1 -> CellCore_in3/9
  UCell10_mV/1 -> CellCore_in3/10
  UCell11_mV/1 -> CellCore_in3/11
  UCell12_mV/1 -> CellCore_in3/12
  UCell13_mV/1 -> CellCore_in3/13
  UCell14_mV/1 -> CellCore_in3/14
  CellCore_in3/1 -> CellCore/3(mV)
  UCell01Qlf/1 -> CellCore_in4/1
  UCell02Qlf/1 -> CellCore_in4/2
  UCell03Qlf/1 -> CellCore_in4/3
  UCell04Qlf/1 -> CellCore_in4/4
  UCell05Qlf/1 -> CellCore_in4/5
  UCell06Qlf/1 -> CellCore_in4/6
  UCell07Qlf/1 -> CellCore_in4/7
  UCell08Qlf/1 -> CellCore_in4/8
  UCell09Qlf/1 -> CellCore_in4/9
  UCell10Qlf/1 -> CellCore_in4/10
  UCell11Qlf/1 -> CellCore_in4/11
  UCell12Qlf/1 -> CellCore_in4/12
  UCell13Qlf/1 -> CellCore_in4/13
  UCell14Qlf/1 -> CellCore_in4/14
  CellCore_in4/1 -> CellCore/4(qlf)
  OutputEnable/1 -> CellCore/5(outEn)
  LimitActive/1 -> CellCore/6(limitActive)
  ControllerOffReq/1 -> CellCore/7(ctrlOffReq)
  CalSetOffset_V_r/1 -> CellCore/8(calSO)
  CalSetGain_r/1 -> CellCore/9(calSG)
  CalMeasOffset_V_r/1 -> CellCore/10(calMO)
  CalMeasGain_r/1 -> CellCore/11(calMG)
  HandActive/1 -> CellCore/12(handOn)
  HandSetpoint_V_r/1 -> CellCore/13(handSp)
  HandEnable_r/1 -> CellCore/14(handEn)
  SelectedChannel/1 -> CellCore/15(selCh)
  SelectAllMode/1 -> CellCore/16(selAll)
  VoltageSetValue_Ax_Const/1 -> CellCore/17(setAx)
  VoltageSetPwm_T_Const/1 -> CellCore/18(setT)
  VoltageSenseMeas_Ax_Const/1 -> CellCore/19(senseAx)
  VoltageSenseValue_T_Const/1 -> CellCore/20(senseT)
  SetpointLimit_V_Const/1 -> CellCore/21(limitV)
  VoltageSenseFilter_Const/1 -> CellCore/22(filt)
  CtrlKp_Const/1 -> CellCore/23(kp)
  CtrlKi_per_s_Const/1 -> CellCore/24(kiPerS)
  CtrlLimit_V_Const/1 -> CellCore/25(ctrlLim)
  OverVoltThd_V_Const/1 -> CellCore/26(ovThd)
  OverVoltTime_cycles_Const/1 -> CellCore/27(ovN)
  OutputFloor_V_Const/1 -> CellCore/28(floorV)
  StepThreshold_V_Const/1 -> CellCore/29(stepThd)
  StepHold_cycles_Const/1 -> CellCore/30(stepN)
  QLF_OK_Const/1 -> CellCore/31(QlfOk)
  CellCore/1(en) -> CellCore_out1/1
  CellCore_out1/1 -> En01/1
  CellCore_out1/2 -> En02/1
  CellCore_out1/3 -> En03/1
  CellCore_out1/4 -> En04/1
  CellCore_out1/5 -> En05/1
  CellCore_out1/6 -> En06/1
  CellCore_out1/7 -> En07/1
  CellCore_out1/8 -> En08/1
  CellCore_out1/9 -> En09/1
  CellCore_out1/10 -> En10/1
  CellCore_out1/11 -> En11/1
  CellCore_out1/12 -> En12/1
  CellCore_out1/13 -> En13/1
  CellCore_out1/14 -> En14/1
  CellCore/2(vAct) -> CellCore_out2/1
  CellCore_out2/1 -> Cell01VoltAct_V/1
  CellCore_out2/2 -> Cell02VoltAct_V/1
  CellCore_out2/3 -> Cell03VoltAct_V/1
  CellCore_out2/4 -> Cell04VoltAct_V/1
  CellCore_out2/5 -> Cell05VoltAct_V/1
  CellCore_out2/6 -> Cell06VoltAct_V/1
  CellCore_out2/7 -> Cell07VoltAct_V/1
  CellCore_out2/8 -> Cell08VoltAct_V/1
  CellCore_out2/9 -> Cell09VoltAct_V/1
  CellCore_out2/10 -> Cell10VoltAct_V/1
  CellCore_out2/11 -> Cell11VoltAct_V/1
  CellCore_out2/12 -> Cell12VoltAct_V/1
  CellCore_out2/13 -> Cell13VoltAct_V/1
  CellCore_out2/14 -> Cell14VoltAct_V/1
  CellCore/3(state) -> CellCore_out3/1
  CellCore_out3/1 -> Cell01State/1
  CellCore_out3/2 -> Cell02State/1
  CellCore_out3/3 -> Cell03State/1
  CellCore_out3/4 -> Cell04State/1
  CellCore_out3/5 -> Cell05State/1
  CellCore_out3/6 -> Cell06State/1
  CellCore_out3/7 -> Cell07State/1
  CellCore_out3/8 -> Cell08State/1
  CellCore_out3/9 -> Cell09State/1
  CellCore_out3/10 -> Cell10State/1
  CellCore_out3/11 -> Cell11State/1
  CellCore_out3/12 -> Cell12State/1
  CellCore_out3/13 -> Cell13State/1
  CellCore_out3/14 -> Cell14State/1
  CellCore/4(duty) -> CellCore_out4/1
  CellCore_out4/1 -> Duty01/1
  CellCore_out4/2 -> Duty02/1
  CellCore_out4/3 -> Duty03/1
  CellCore_out4/4 -> Duty04/1
  CellCore_out4/5 -> Duty05/1
  CellCore_out4/6 -> Duty06/1
  CellCore_out4/7 -> Duty07/1
  CellCore_out4/8 -> Duty08/1
  CellCore_out4/9 -> Duty09/1
  CellCore_out4/10 -> Duty10/1
  CellCore_out4/11 -> Duty11/1
  CellCore_out4/12 -> Duty12/1
  CellCore_out4/13 -> Duty13/1
  CellCore_out4/14 -> Duty14/1
  CellCore/5(ctrlOn) -> ControllerOn/1
  CellCore/6(ctrlOffAct) -> ControllerOffAct/1
  CellCore/7(overVolt) -> OverVoltage/1
  CellCore/8(released) -> ChannelsReleased/1
  CellCore/9(selLed) -> CellCore_out9/1
  CellCore_out9/1 -> Sel01/1
  CellCore_out9/2 -> Sel02/1
  CellCore_out9/3 -> Sel03/1
  CellCore_out9/4 -> Sel04/1
  CellCore_out9/5 -> Sel05/1
  CellCore_out9/6 -> Sel06/1
  CellCore_out9/7 -> Sel07/1
  CellCore_out9/8 -> Sel08/1
  CellCore_out9/9 -> Sel09/1
  CellCore_out9/10 -> Sel10/1
  CellCore_out9/11 -> Sel11/1
  CellCore_out9/12 -> Sel12/1
  CellCore_out9/13 -> Sel13/1
  CellCore_out9/14 -> Sel14/1
  CellCore/10(actOut) -> ActualVolt_V_r/1
  Cell15State_Const/1 -> Cell15State/1
  Cell16State_Const/1 -> Cell16State/1
  Cell15VoltAct_V_Default/1 -> Cell15VoltAct_V/1
  Cell16VoltAct_V_Default/1 -> Cell16VoltAct_V/1

== matlab function CellChannels/CellChannels_task10ms/CellCore ==
  data: setV input; en output; enable input; mV input; qlf input; outEn input; limitActive input; ctrlOffReq input; calSO input; calSG input; calMO input; calMG input; handOn input; handSp input; handEn input; selCh input; selAll input; setAx input; setT input; senseAx input; senseT input; limitV input; filt input; kp input; kiPerS input; ctrlLim input; ovThd input; ovN input; floorV input; stepThd input; stepN input; QlfOk input; vAct output; state output; duty output; ctrlOn output; ctrlOffAct output; overVolt output; released output; selLed output; actOut output
function [en, vAct, state, duty, ctrlOn, ctrlOffAct, overVolt, released, selLed, actOut] = CellCore(setV, enable, mV, qlf, outEn, limitActive, ctrlOffReq, ...
    calSO, calSG, calMO, calMG, handOn, handSp, handEn, selCh, selAll, setAx, setT, senseAx, senseT, limitV, filt, kp, kiPerS, ctrlLim, ovThd, ovN, floorV, stepThd, stepN, QlfOk)
%CELLCORE 14 cell channels: setpoint -> duty, release, actual value, regulator, status (see CellChannels_create.m).
%#codegen
persistent y seen integ corrHold ovCnt prevV holdCnt
if isempty(y)
    y = zeros(14, 1, 'single');
    seen = false(14, 1);
    integ = zeros(14, 1, 'single');
    corrHold = zeros(14, 1, 'single');
    ovCnt = zeros(14, 1, 'uint8');      % samples in a row above setpoint + threshold
    prevV = zeros(14, 1, 'single');     % limited setpoint of the previous step
    holdCnt = zeros(14, 1, 'uint8');    % regulator hold after a setpoint step
end
en = false(14, 1);
vAct = zeros(14, 1, 'single');
state = zeros(14, 1, 'uint8');
duty = zeros(14, 1, 'uint16');
ctrlActive = (ctrlOffReq == uint8(0));
ctrlOn = ctrlActive;
ctrlOffAct = uint8(ctrlOffReq ~= uint8(0));
ts = single(0.01);
for k = 1:14
    if handOn
        commanded = handEn(k);
        v = handSp(k);
    else
        commanded = (enable(k) == uint8(2));
        v = setV(k);
    end
    clipped = (v > limitV);
    if clipped
        v = limitV;
    end
    if ~(v > single(0))
        v = single(0);
    end
    below = commanded && (v > single(0)) && (v < floorV) && ~clipped;
    if abs(v - prevV(k)) > stepThd
        holdCnt(k) = stepN;
    end
    prevV(k) = v;
    holding = holdCnt(k) > uint8(0);
    if holding
        holdCnt(k) = holdCnt(k) - uint8(1);
    end
    [sg, so] = plausible(calSG(k), calSO(k));
    [mg, mo] = plausible(calMG(k), calMO(k));
    % actual value: curve, calibration, low-pass
    if qlf(k) == QlfOk
        mv = mg * interp1d(senseAx, senseT, single(mV(k))) + mo;
        if outEn && commanded && (mv - max(v, floorV) > ovThd)
            if ovCnt(k) < uint8(255)
                ovCnt(k) = ovCnt(k) + uint8(1);
            end
        else
            ovCnt(k) = uint8(0);
        end
        if seen(k)
            y(k) = y(k) + filt * (mv - y(k));
        else
            y(k) = mv;
            seen(k) = true;
        end
    end
    vAct(k) = y(k);
    if ~(outEn && commanded)
        ovCnt(k) = uint8(0);
    end
    % regulator: PI on the actual value, correction limited, integral part clamped (anti-windup)
    corr = single(0);
    working = ctrlActive && outEn && commanded && ~clipped && (v > single(0)) && ~below && (qlf(k) == QlfOk) && seen(k);
    if holding
        integ(k) = single(0);              % setpoint step: correction and integral part 0, held at 0 for the hold time
        corrHold(k) = single(0);
    elseif working && limitActive
        corr = corrHold(k);                % LIMIT of the supply: stand still
    elseif working
        e = v - y(k);
        iNew = integ(k) + kiPerS * ts * e;
        iNew = min(max(iNew, -ctrlLim), ctrlLim);
        integ(k) = iNew;
        corr = min(max(kp * e + iNew, -ctrlLim), ctrlLim);
        corrHold(k) = corr;
    else
        integ(k) = single(0);
        corrHold(k) = single(0);
    end
    % setpoint -> command -> duty
    if outEn && commanded && (v > single(0))
        cmd = min(max(v + corr, single(0)), limitV);
        cmd = sg * cmd + so;
        d = interp1d(setAx, setT, cmd) * single(10000);
        d = min(max(d, single(0)), single(10000));
        duty(k) = uint16(floor(d + single(0.5)));
    end
    en(k) = outEn && commanded;
    if ~commanded
        state(k) = uint8(1);
    elseif clipped
        state(k) = uint8(3);
    elseif below
        state(k) = uint8(4);
    else
        state(k) = uint8(2);
    end
end
selLed = false(14, 1);
if handOn
    for k = 1:14
        selLed(k) = selAll || (uint8(k) == selCh);
    end
end
actOut = vAct;
released = any(en);
overVolt = any(ovCnt >= ovN);      % one assignment after the loop: an accumulating output would read the RTE write call

function [g, o] = plausible(gain, offset)
% a calibration pair outside 0.5 .. 1.5 / +-0.5 V (CellCal never delivers one; the port is 0 before its first run) is the factory value
g = gain;
o = offset;
if ~((gain >= single(0.5)) && (gain <= single(1.5)) && (abs(offset) <= single(0.5)))
    g = single(1);
    o = single(0);
end

function y = interp1d(ax, tab, v)
% linear interpolation, constant outside the breakpoints
n = numel(ax);
y = tab(n);
if v <= ax(1)
    y = tab(1);
else
    for i = 1:n - 1
        if v <= ax(i + 1)
            y = tab(i) + (tab(i + 1) - tab(i)) * (v - ax(i)) / (ax(i + 1) - ax(i));
            break;
        end
    end
end
